simulink model "lqr_observer_drone"  (R2026a)
settings: Solver=ode15s  StopTime=2
values from neighbouring files (symbols this model uses):
  B = sys.B    [eigenvalue_placement.m]    (also in linear_system.m = zeros(14,4); lqr_controller.m; lqr_with_observer.m)
  K = zeros(m, n)    [eigenvalue_placement.m]    (also in eigval_controller.mat = [0 0 -3.3747905109 0 0 -3.41929470324 0 0 45.8010025 0 0 0 .; lqr_controller.mat = [-2.73545264692e-15 4.11267675522e-14 -14.1421356237 -6.3332; lqr_with_observer.m = lqr(A, B, Q_lqr, R_lqr))
  L = place(A', C', observer_poles)'    [lqr_with_observer.m]
  U = -(K*(X - xref.').').'    [eigenvalue_placement.m]
  x0 = zeros(n,1)    [eigenvalue_placement.m]    (also in lqr_controller.m = ones(n, 1); lqr_with_observer.m = ones(n, 1))
undefined symbols (not defined in the file or in its folder): xhat0
settings Model: Creator=shrey  LastModifiedBy=vibhakamath

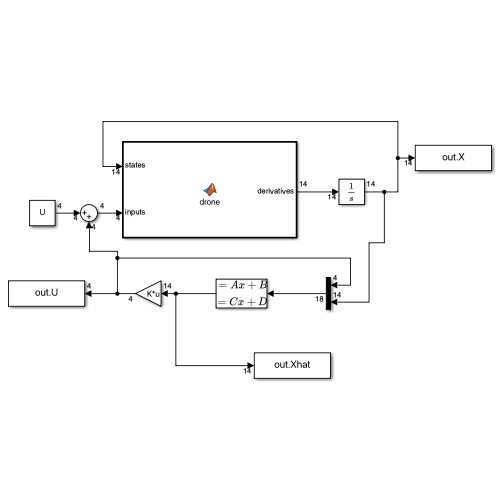
[thumbnail: Simulink's stored preview of the top-level diagram]
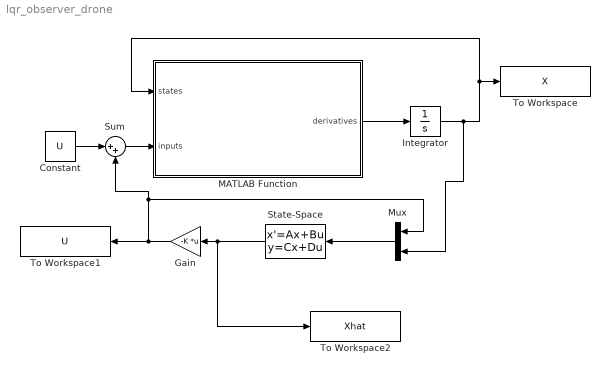
== system lqr_observer_drone ==
  Constant : Constant  Value=U
  Gain : Gain  Gain=-K  Multiplication=Matrix(K*u)
  Integrator : Integrator  InitialCondition=x0
  MATLAB Function : MATLAB Function  TreatAsAtomicUnit=on
  Mux : Mux  Inputs=2
  State-Space : StateSpace  A=A - L  B=[B L]  C=eye(14)  D=zeros(14, 18)  InitialCondition=xhat0
  Sum : Sum  Inputs=|++
  To Workspace : ToWorkspace  VariableName=X  SampleTime=-1
  To Workspace1 : ToWorkspace  VariableName=U  SampleTime=-1
  To Workspace2 : ToWorkspace  VariableName=Xhat  SampleTime=-1
  wires:
  Integrator/1 -> Mux/2, To Workspace/1, MATLAB Function/1(states)
  Constant/1 -> Sum/1
  Sum/1 -> MATLAB Function/2(inputs)
  MATLAB Function/1(derivatives) -> Integrator/1
  State-Space/1 -> To Workspace2/1, Gain/1
  Gain/1 -> Mux/1, Sum/2, To Workspace1/1
  Mux/1 -> State-Space/1

== matlab function lqr_observer_drone/MATLAB Function ==
  data: states input; derivatives output; inputs input; parameters parameter
function derivatives = drone(states, inputs, parameters)

    zeta     = states(1:3);
    zeta_dot = states(4:6);
    x_dot = zeta_dot(1);
    y_dot = zeta_dot(2);
    z_dot = zeta_dot(3);

    phi   = states(7);
    theta = states(8);
    psi   = states(9);

    p = states(10);
    q = states(11);
    r = states(12);

    alpha     = states(13);
    alpha_dot = states(14);

    u_tot   = inputs(1);   % total thrust
    u_phi   = inputs(2);   % torques
    u_theta = inputs(3);
    u_psi   = inputs(4);

    Fx = (cos(psi) * sin(theta) * cos(phi) + sin(psi) * sin(phi)) * u_tot;
    Fy = (sin(psi) * sin(theta) * cos(phi) - cos(psi) * sin(phi)) * u_tot;
    Fz = (cos(theta) * cos(phi)) * u_tot;

    g   = parameters.g;
    m   = parameters.m;
    mp  = parameters.mp;
    M   = m + mp;
    Ixx = parameters.Ixx;
    Iyy = parameters.Iyy;
    Izz = parameters.Izz;
    kD  = parameters.kD;
    l   = parameters.l;

    x_dot_d = ((m + mp * cos(alpha)^2) * (Fx - kD * x_dot) ...
              - mp * sin(alpha) * cos(alpha) * (Fz - kD * z_dot) ...
              + m * mp * l * alpha_dot^2 * sin(alpha)) / (m * M);
    y_dot_d = (Fy - kD * y_dot) / m;
    z_dot_d = ((m + mp * sin(alpha)^2) * (Fz - kD * z_dot) ...
              - mp * sin(alpha) * cos(alpha) * (Fx - kD * x_dot) ...
              + m * mp * l * alpha_dot^2 * cos(alpha)) / (m * M) - g;

    phi_dot   = p + q * sin(phi) * tan(theta) + r * cos(phi) * tan(theta);
    theta_dot = q * cos(phi) - r * sin(phi);
    psi_dot   = (q * sin(phi) + r * cos(phi)) / cos(theta);

    p_dot = u_phi   / Ixx + (Iyy - Izz) / Ixx * q * r;
    q_dot = u_theta / Iyy + (Izz - Ixx) / Iyy * p * r;
    r_dot = u_psi   / Izz + (Ixx - Iyy) / Izz * p * q;

    alpha_dot_d = (-Fx * cos(alpha) + Fz * sin(alpha) ...
                   + kD * x_dot * cos(alpha) - kD * z_dot * sin(alpha)) / (M * l);

    derivatives = [zeta_dot;
                   x_dot_d; y_dot_d; z_dot_d;
                   phi_dot; theta_dot; psi_dot;
                   p_dot; q_dot; r_dot;
                   alpha_dot;
                   alpha_dot_d];
end
